simulink model "Bench_Live"  (R2026b)
settings: Solver=ode1  StopTime=inf  FixedStep=Ts
undefined symbols (not defined in the file): du_min, ISCS_Ad, ISCS_Bd, ISCS_Cd, ISCS_Dd, ISCS_Tu, ISCS_Ty, P_on, Ts
settings Model: Creator=williamvandevoir  LastModifiedBy=leont

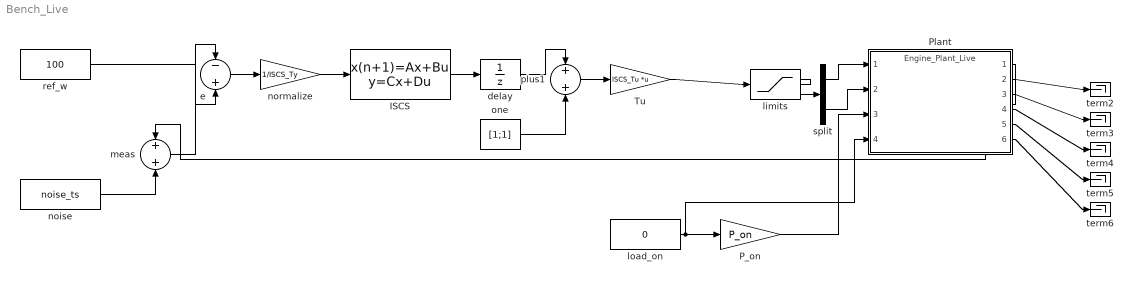
== system Bench_Live ==
  ISCS : DiscreteStateSpace  A=ISCS_Ad  B=ISCS_Bd  C=ISCS_Cd  D=ISCS_Dd  InitialCondition=zeros(12,1)  SampleTime=Ts
  P_on : Gain  Gain=P_on
  Plant : ModelReference  ModelNameDialog=Engine_Plant_Live  SimulationMode=Normal  ModelReferenceVersion=1.25
  Tu : Gain  Gain=ISCS_Tu  Multiplication=Matrix(K*u)
  delay : UnitDelay  InitialCondition=zeros(2,1)  SampleTime=Ts
  e : Sum  Inputs=-+
  limits : Saturate  UpperLimit=[100; 0]  LowerLimit=[0; du_min]
  load_on : Constant  Value=0
  meas : Sum
  noise : FromWorkspace  VariableName=noise_ts  SampleTime=Ts  Interpolate=off  OutputAfterFinalValue=Cyclic repetition
  normalize : Gain  Gain=1/ISCS_Ty
  one : Constant  Value=[1;1]
  plus1 : Sum
  ref_w : Constant  Value=100
  split : Demux  Outputs=2
  term{2..6} (5 alike) : Terminator
  wires:
  ref_w/1 -> e/2
  Plant/1 -> meas/1
  noise/1 -> meas/2
  meas/1 -> e/1
  e/1 -> normalize/1
  normalize/1 -> ISCS/1
  ISCS/1 -> delay/1
  delay/1 -> plus1/1
  one/1 -> plus1/2
  plus1/1 -> Tu/1
  limits/1 -> split/1
  split/1 -> Plant/1
  split/2 -> Plant/2
  load_on/1 -> P_on/1, Plant/4
  P_on/1 -> Plant/3
  Plant/2 -> term2/1
  Plant/3 -> term3/1
  Plant/4 -> term4/1
  Plant/5 -> term5/1
  Plant/6 -> term6/1
  Tu/1 -> limits/1
